simulink model "rfsoc4x2_ospfb_128"  (R2021a)
settings: Solver=VariableStepAuto  StartTime=0.0  StopTime=2048  RelTol=1e-3
undefined symbols (not defined in the file): pfb_coeff_gen_calc
libraries: xbsIndex_r4 x25898, casper_library_delays x113, casper_library_misc x68, xps_library x1
(part 83 of 221)

== system rfsoc4x2_ospfb_128/fft_wideband_real/fft_unscrambler/reorder/buf5 ==
  addr : Inport
  din : Inport  Port=2
  we : Inport  Port=3
  bram0 : xbsIndex_r4/Single Port RAM  depth=16  initVector=getfield(get_param(gcb, 'UserData'), 'initVector')  distributed_mem=Block RAM  write_mode=Read Before Write  rst=off  init_reg=0  en=off  optimize_latency=off  latency=3  optimize=Speed  dbl_ovrd=off  simulation_type=fast_sim  block_type=spram
  ddin : xbsIndex_r4/Delay  rst=off  infoeditControl=Selection of Reset will increase slice count due to use of real FFs and instead of SRLs  en=off  latency=0  reg_retiming=on  dbl_ovrd=off  block_type=delay
  debus_addr : Subsystem  AncestorBlock=casper_library_flow_control/bus_expand  mask(bus_expand){mode=divisions of equal size, outputNum=1, outputWidth=4, outputBinaryPt=0, outputArithmeticType=0, show_format=on, outputToWorkspace=off, variablePrefix=, outputToModelAsWell=on}
      mask prompts: outputNum "Number of outputs:"; outputWidth "Output width:"; outputBinaryPt "Output binary point position:"; outputArithmeticType "Output arithmetic type (ufix=0, fix=1, bool=2):"; show_format "Print format string?"; outputToWorkspace "Output to workspace?"; variablePrefix "Variable name prefix:"; outputToModelAsWell "Output to model as well?"
      mask help:
      | Expands a 'bus' made using a bus_create or Xilinx
      | concat block.
      | The input will be divided into the specified number
      | of outputs with the specified arithmetic types.
      | Divisions are made from most significant bit.
      mask init: same as rfsoc4x2_ospfb_128/bus_expand
      settings: AttributesFormatString=1 outputs: uf4.0,
      mask TypeOptions mode: divisions of equal size | divisions of arbitrary size
      mask Callback mode: %bus_expand_callback();
      mask Callback outputWidth: %bus_expand_callback();
      mask Callback outputToWorkspace: %bus_expand_callback();
  debus_din : Subsystem  AncestorBlock=casper_library_flow_control/bus_expand  mask(bus_expand){mode=divisions of arbitrary size, outputNum=2, outputWidth=36, outputBinaryPt=0, outputArithmeticType=0, show_format=on, outputToWorkspace=off, variablePrefix=, outputToModelAsWell=on}
      mask prompts: outputNum "Number of outputs:"; outputWidth "Output width:"; outputBinaryPt "Output binary point position:"; outputArithmeticType "Output arithmetic type (ufix=0, fix=1, bool=2):"; show_format "Print format string?"; outputToWorkspace "Output to workspace?"; variablePrefix "Variable name prefix:"; outputToModelAsWell "Output to model as well?"
      mask help:
      | Expands a 'bus' made using a bus_create or Xilinx
      | concat block.
      | The input will be divided into the specified number
      | of outputs with the specified arithmetic types.
      | Divisions are made from most significant bit.
      mask init: same as rfsoc4x2_ospfb_128/bus_expand
      settings: AttributesFormatString=1 outputs: uf36.0,
      mask TypeOptions mode: divisions of equal size | divisions of arbitrary size
      mask Callback mode: %bus_expand_callback();
      mask Callback outputWidth: %bus_expand_callback();
      mask Callback outputToWorkspace: %bus_expand_callback();
  debus_we : Subsystem  AncestorBlock=casper_library_flow_control/bus_expand  mask(bus_expand){mode=divisions of equal size, outputNum=1, outputWidth=1, outputBinaryPt=0, outputArithmeticType=2, show_format=on, outputToWorkspace=off, variablePrefix=, outputToModelAsWell=on}
      mask prompts: outputNum "Number of outputs:"; outputWidth "Output width:"; outputBinaryPt "Output binary point position:"; outputArithmeticType "Output arithmetic type (ufix=0, fix=1, bool=2):"; show_format "Print format string?"; outputToWorkspace "Output to workspace?"; variablePrefix "Variable name prefix:"; outputToModelAsWell "Output to model as well?"
      mask help:
      | Expands a 'bus' made using a bus_create or Xilinx
      | concat block.
      | The input will be divided into the specified number
      | of outputs with the specified arithmetic types.
      | Divisions are made from most significant bit.
      mask init: same as rfsoc4x2_ospfb_128/bus_expand
      settings: AttributesFormatString=1 outputs: b,
      mask TypeOptions mode: divisions of equal size | divisions of arbitrary size
      mask Callback mode: %bus_expand_callback();
      mask Callback outputWidth: %bus_expand_callback();
      mask Callback outputToWorkspace: %bus_expand_callback();
  din_bussify : Subsystem  AncestorBlock=casper_library_flow_control/bus_create  mask(bus_create){inputNum=1}
      mask prompts: inputNum "Number of inputs:"
      mask init:
      | bus_create_init(gcb,...
      |     'inputNum', inputNum);
  rep_addr : Subsystem  AncestorBlock=casper_library_bus/bus_replicate  mask(bus_replicate){replication=1, csp_latency=0, misc=off, implementation=core}
      mask prompts: replication "replication factor"; csp_latency "latency"; misc "misc support"; implementation "delay implementation"
      mask help: Output bus formed by replicating input bus a number of times
      mask init:
      | bus_replicate_init(gcb, ...
      |     'replication', replication, ...
      |     'csp_latency', csp_latency, ...
      |     'implementation', implementation, ...
      |     'misc', misc);
      mask TypeOptions implementation: core | behavioral
  rep_we : Subsystem  AncestorBlock=casper_library_bus/bus_replicate  mask(bus_replicate){replication=1, csp_latency=0, misc=off, implementation=core}
      mask prompts: replication "replication factor"; csp_latency "latency"; misc "misc support"; implementation "delay implementation"
      mask help: Output bus formed by replicating input bus a number of times
      mask init:
      | bus_replicate_init(gcb, ...
      |     'replication', replication, ...
      |     'csp_latency', csp_latency, ...
      |     'implementation', implementation, ...
      |     'misc', misc);
      mask TypeOptions implementation: core | behavioral
  dout : Outport
  wires:
  addr/1 -> rep_addr/1(in)
  din/1 -> ddin/1
  we/1 -> rep_we/1(in)
  rep_addr/1(out) -> debus_addr/1(bus_in)
  ddin/1 -> debus_din/1(bus_in)
  rep_we/1(out) -> debus_we/1(bus_in)
  debus_addr/1(msb_lsb_out1) -> bram0/1
  debus_din/1(msb_lsb_out1) -> bram0/2
  debus_we/1(msb_lsb_out1) -> bram0/3
  bram0/1 -> din_bussify/1(in1)
  din_bussify/1(bus_out) -> dout/1

== system rfsoc4x2_ospfb_128/fft_wideband_real/fft_unscrambler/reorder/buf6 ==
  addr : Inport
  din : Inport  Port=2
  we : Inport  Port=3
  bram0 : xbsIndex_r4/Single Port RAM  depth=16  initVector=getfield(get_param(gcb, 'UserData'), 'initVector')  distributed_mem=Block RAM  write_mode=Read Before Write  rst=off  init_reg=0  en=off  optimize_latency=off  latency=3  optimize=Speed  dbl_ovrd=off  simulation_type=fast_sim  block_type=spram
  ddin : xbsIndex_r4/Delay  rst=off  infoeditControl=Selection of Reset will increase slice count due to use of real FFs and instead of SRLs  en=off  latency=0  reg_retiming=on  dbl_ovrd=off  block_type=delay
  debus_addr : Subsystem  AncestorBlock=casper_library_flow_control/bus_expand  mask(bus_expand){mode=divisions of equal size, outputNum=1, outputWidth=4, outputBinaryPt=0, outputArithmeticType=0, show_format=on, outputToWorkspace=off, variablePrefix=, outputToModelAsWell=on}
      mask prompts: outputNum "Number of outputs:"; outputWidth "Output width:"; outputBinaryPt "Output binary point position:"; outputArithmeticType "Output arithmetic type (ufix=0, fix=1, bool=2):"; show_format "Print format string?"; outputToWorkspace "Output to workspace?"; variablePrefix "Variable name prefix:"; outputToModelAsWell "Output to model as well?"
      mask help:
      | Expands a 'bus' made using a bus_create or Xilinx
      | concat block.
      | The input will be divided into the specified number
      | of outputs with the specified arithmetic types.
      | Divisions are made from most significant bit.
      mask init: same as rfsoc4x2_ospfb_128/bus_expand
      settings: AttributesFormatString=1 outputs: uf4.0,
      mask TypeOptions mode: divisions of equal size | divisions of arbitrary size
      mask Callback mode: %bus_expand_callback();
      mask Callback outputWidth: %bus_expand_callback();
      mask Callback outputToWorkspace: %bus_expand_callback();
  debus_din : Subsystem  AncestorBlock=casper_library_flow_control/bus_expand  mask(bus_expand){mode=divisions of arbitrary size, outputNum=2, outputWidth=36, outputBinaryPt=0, outputArithmeticType=0, show_format=on, outputToWorkspace=off, variablePrefix=, outputToModelAsWell=on}
      mask prompts: outputNum "Number of outputs:"; outputWidth "Output width:"; outputBinaryPt "Output binary point position:"; outputArithmeticType "Output arithmetic type (ufix=0, fix=1, bool=2):"; show_format "Print format string?"; outputToWorkspace "Output to workspace?"; variablePrefix "Variable name prefix:"; outputToModelAsWell "Output to model as well?"
      mask help:
      | Expands a 'bus' made using a bus_create or Xilinx
      | concat block.
      | The input will be divided into the specified number
      | of outputs with the specified arithmetic types.
      | Divisions are made from most significant bit.
      mask init: same as rfsoc4x2_ospfb_128/bus_expand
      settings: AttributesFormatString=1 outputs: uf36.0,
      mask TypeOptions mode: divisions of equal size | divisions of arbitrary size
      mask Callback mode: %bus_expand_callback();
      mask Callback outputWidth: %bus_expand_callback();
      mask Callback outputToWorkspace: %bus_expand_callback();
  debus_we : Subsystem  AncestorBlock=casper_library_flow_control/bus_expand  mask(bus_expand){mode=divisions of equal size, outputNum=1, outputWidth=1, outputBinaryPt=0, outputArithmeticType=2, show_format=on, outputToWorkspace=off, variablePrefix=, outputToModelAsWell=on}
      mask prompts: outputNum "Number of outputs:"; outputWidth "Output width:"; outputBinaryPt "Output binary point position:"; outputArithmeticType "Output arithmetic type (ufix=0, fix=1, bool=2):"; show_format "Print format string?"; outputToWorkspace "Output to workspace?"; variablePrefix "Variable name prefix:"; outputToModelAsWell "Output to model as well?"
      mask help:
      | Expands a 'bus' made using a bus_create or Xilinx
      | concat block.
      | The input will be divided into the specified number
      | of outputs with the specified arithmetic types.
      | Divisions are made from most significant bit.
      mask init: same as rfsoc4x2_ospfb_128/bus_expand
      settings: AttributesFormatString=1 outputs: b,
      mask TypeOptions mode: divisions of equal size | divisions of arbitrary size
      mask Callback mode: %bus_expand_callback();
      mask Callback outputWidth: %bus_expand_callback();
      mask Callback outputToWorkspace: %bus_expand_callback();
  din_bussify : Subsystem  AncestorBlock=casper_library_flow_control/bus_create  mask(bus_create){inputNum=1}
      mask prompts: inputNum "Number of inputs:"
      mask init:
      | bus_create_init(gcb,...
      |     'inputNum', inputNum);
  rep_addr : Subsystem  AncestorBlock=casper_library_bus/bus_replicate  mask(bus_replicate){replication=1, csp_latency=0, misc=off, implementation=core}
      mask prompts: replication "replication factor"; csp_latency "latency"; misc "misc support"; implementation "delay implementation"
      mask help: Output bus formed by replicating input bus a number of times
      mask init:
      | bus_replicate_init(gcb, ...
      |     'replication', replication, ...
      |     'csp_latency', csp_latency, ...
      |     'implementation', implementation, ...
      |     'misc', misc);
      mask TypeOptions implementation: core | behavioral
  rep_we : Subsystem  AncestorBlock=casper_library_bus/bus_replicate  mask(bus_replicate){replication=1, csp_latency=0, misc=off, implementation=core}
      mask prompts: replication "replication factor"; csp_latency "latency"; misc "misc support"; implementation "delay implementation"
      mask help: Output bus formed by replicating input bus a number of times
      mask init:
      | bus_replicate_init(gcb, ...
      |     'replication', replication, ...
      |     'csp_latency', csp_latency, ...
      |     'implementation', implementation, ...
      |     'misc', misc);
      mask TypeOptions implementation: core | behavioral
  dout : Outport
  wires:
  addr/1 -> rep_addr/1(in)
  din/1 -> ddin/1
  we/1 -> rep_we/1(in)
  rep_addr/1(out) -> debus_addr/1(bus_in)
  ddin/1 -> debus_din/1(bus_in)
  rep_we/1(out) -> debus_we/1(bus_in)
  debus_addr/1(msb_lsb_out1) -> bram0/1
  debus_din/1(msb_lsb_out1) -> bram0/2
  debus_we/1(msb_lsb_out1) -> bram0/3
  bram0/1 -> din_bussify/1(in1)
  din_bussify/1(bus_out) -> dout/1

== system rfsoc4x2_ospfb_128/fft_wideband_real/fft_unscrambler/reorder/buf7 ==
  addr : Inport
  din : Inport  Port=2
  we : Inport  Port=3
  bram0 : xbsIndex_r4/Single Port RAM  depth=16  initVector=getfield(get_param(gcb, 'UserData'), 'initVector')  distributed_mem=Block RAM  write_mode=Read Before Write  rst=off  init_reg=0  en=off  optimize_latency=off  latency=3  optimize=Speed  dbl_ovrd=off  simulation_type=fast_sim  block_type=spram
  ddin : xbsIndex_r4/Delay  rst=off  infoeditControl=Selection of Reset will increase slice count due to use of real FFs and instead of SRLs  en=off  latency=0  reg_retiming=on  dbl_ovrd=off  block_type=delay
  debus_addr : Subsystem  AncestorBlock=casper_library_flow_control/bus_expand  mask(bus_expand){mode=divisions of equal size, outputNum=1, outputWidth=4, outputBinaryPt=0, outputArithmeticType=0, show_format=on, outputToWorkspace=off, variablePrefix=, outputToModelAsWell=on}
      mask prompts: outputNum "Number of outputs:"; outputWidth "Output width:"; outputBinaryPt "Output binary point position:"; outputArithmeticType "Output arithmetic type (ufix=0, fix=1, bool=2):"; show_format "Print format string?"; outputToWorkspace "Output to workspace?"; variablePrefix "Variable name prefix:"; outputToModelAsWell "Output to model as well?"
      mask help:
      | Expands a 'bus' made using a bus_create or Xilinx
      | concat block.
      | The input will be divided into the specified number
      | of outputs with the specified arithmetic types.
      | Divisions are made from most significant bit.
      mask init: same as rfsoc4x2_ospfb_128/bus_expand
      settings: AttributesFormatString=1 outputs: uf4.0,
      mask TypeOptions mode: divisions of equal size | divisions of arbitrary size
      mask Callback mode: %bus_expand_callback();
      mask Callback outputWidth: %bus_expand_callback();
      mask Callback outputToWorkspace: %bus_expand_callback();
  debus_din : Subsystem  AncestorBlock=casper_library_flow_control/bus_expand  mask(bus_expand){mode=divisions of arbitrary size, outputNum=2, outputWidth=36, outputBinaryPt=0, outputArithmeticType=0, show_format=on, outputToWorkspace=off, variablePrefix=, outputToModelAsWell=on}
      mask prompts: outputNum "Number of outputs:"; outputWidth "Output width:"; outputBinaryPt "Output binary point position:"; outputArithmeticType "Output arithmetic type (ufix=0, fix=1, bool=2):"; show_format "Print format string?"; outputToWorkspace "Output to workspace?"; variablePrefix "Variable name prefix:"; outputToModelAsWell "Output to model as well?"
      mask help:
      | Expands a 'bus' made using a bus_create or Xilinx
      | concat block.
      | The input will be divided into the specified number
      | of outputs with the specified arithmetic types.
      | Divisions are made from most significant bit.
      mask init: same as rfsoc4x2_ospfb_128/bus_expand
      settings: AttributesFormatString=1 outputs: uf36.0,
      mask TypeOptions mode: divisions of equal size | divisions of arbitrary size
      mask Callback mode: %bus_expand_callback();
      mask Callback outputWidth: %bus_expand_callback();
      mask Callback outputToWorkspace: %bus_expand_callback();
  debus_we : Subsystem  AncestorBlock=casper_library_flow_control/bus_expand  mask(bus_expand){mode=divisions of equal size, outputNum=1, outputWidth=1, outputBinaryPt=0, outputArithmeticType=2, show_format=on, outputToWorkspace=off, variablePrefix=, outputToModelAsWell=on}
      mask prompts: outputNum "Number of outputs:"; outputWidth "Output width:"; outputBinaryPt "Output binary point position:"; outputArithmeticType "Output arithmetic type (ufix=0, fix=1, bool=2):"; show_format "Print format string?"; outputToWorkspace "Output to workspace?"; variablePrefix "Variable name prefix:"; outputToModelAsWell "Output to model as well?"
      mask help:
      | Expands a 'bus' made using a bus_create or Xilinx
      | concat block.
      | The input will be divided into the specified number
      | of outputs with the specified arithmetic types.
      | Divisions are made from most significant bit.
      mask init: same as rfsoc4x2_ospfb_128/bus_expand
      settings: AttributesFormatString=1 outputs: b,
      mask TypeOptions mode: divisions of equal size | divisions of arbitrary size
      mask Callback mode: %bus_expand_callback();
      mask Callback outputWidth: %bus_expand_callback();
      mask Callback outputToWorkspace: %bus_expand_callback();
  din_bussify : Subsystem  AncestorBlock=casper_library_flow_control/bus_create  mask(bus_create){inputNum=1}
      mask prompts: inputNum "Number of inputs:"
      mask init:
      | bus_create_init(gcb,...
      |     'inputNum', inputNum);
  rep_addr : Subsystem  AncestorBlock=casper_library_bus/bus_replicate  mask(bus_replicate){replication=1, csp_latency=0, misc=off, implementation=core}
      mask prompts: replication "replication factor"; csp_latency "latency"; misc "misc support"; implementation "delay implementation"
      mask help: Output bus formed by replicating input bus a number of times
      mask init:
      | bus_replicate_init(gcb, ...
      |     'replication', replication, ...
      |     'csp_latency', csp_latency, ...
      |     'implementation', implementation, ...
      |     'misc', misc);
      mask TypeOptions implementation: core | behavioral
  rep_we : Subsystem  AncestorBlock=casper_library_bus/bus_replicate  mask(bus_replicate){replication=1, csp_latency=0, misc=off, implementation=core}
      mask prompts: replication "replication factor"; csp_latency "latency"; misc "misc support"; implementation "delay implementation"
      mask help: Output bus formed by replicating input bus a number of times
      mask init:
      | bus_replicate_init(gcb, ...
      |     'replication', replication, ...
      |     'csp_latency', csp_latency, ...
      |     'implementation', implementation, ...
      |     'misc', misc);
      mask TypeOptions implementation: core | behavioral
  dout : Outport
  wires:
  addr/1 -> rep_addr/1(in)
  din/1 -> ddin/1
  we/1 -> rep_we/1(in)
  rep_addr/1(out) -> debus_addr/1(bus_in)
  ddin/1 -> debus_din/1(bus_in)
  rep_we/1(out) -> debus_we/1(bus_in)
  debus_addr/1(msb_lsb_out1) -> bram0/1
  debus_din/1(msb_lsb_out1) -> bram0/2
  debus_we/1(msb_lsb_out1) -> bram0/3
  bram0/1 -> din_bussify/1(in1)
  din_bussify/1(bus_out) -> dout/1

== system rfsoc4x2_ospfb_128/fft_wideband_real/fft_unscrambler/reorder/current_map ==
  addra : Inport
  dina : Inport  Port=2
  wea : Inport  Port=3
  addrb : Inport  Port=4
  dinb : Inport  Port=5
  web : Inport  Port=6
  A_bussify0 : Subsystem  AncestorBlock=casper_library_flow_control/bus_create  mask(bus_create){inputNum=1}
      mask prompts: inputNum "Number of inputs:"
      mask init:
      | bus_create_init(gcb,...
      |     'inputNum', inputNum);
  B_bussify0 : Subsystem  AncestorBlock=casper_library_flow_control/bus_create  mask(bus_create){inputNum=1}
      mask prompts: inputNum "Number of inputs:"
      mask init:
      | bus_create_init(gcb,...
      |     'inputNum', inputNum);
  alsbs_slice : xbsIndex_r4/Slice  nbits=4  boolean_output=off  mode=Lower Bit Location + Width  bit1=0  base1=LSB of Input  bit0=0  base0=LSB of Input  dbl_ovrd=off  block_type=slice
  blsbs_slice : xbsIndex_r4/Slice  nbits=4  boolean_output=off  mode=Lower Bit Location + Width  bit1=0  base1=LSB of Input  bit0=0  base0=LSB of Input  dbl_ovrd=off  block_type=slice
  bram0_0 : xbsIndex_r4/Dual Port RAM  depth=16  initVector=getfield(get_param(gcb, 'UserData'), 'initVector')  distributed_mem=Block RAM  init_a=0  init_b=0  rst_a=off  rst_b=off  en_a=off  en_b=off  latency=2  write_mode_A=Read Before Write  write_mode_B=Read Before Write  optimize=Speed  dbl_ovrd=off  simulation_type=fast_sim  block_type=dpram
  ddina0 : xbsIndex_r4/Delay  rst=off  infoeditControl=Selection of Reset will increase slice count due to use of real FFs and instead of SRLs  en=off  latency=0  reg_retiming=on  dbl_ovrd=off  block_type=delay
  ddinb0 : xbsIndex_r4/Delay  rst=off  infoeditControl=Selection of Reset will increase slice count due to use of real FFs and instead of SRLs  en=off  latency=0  reg_retiming=on  dbl_ovrd=off  block_type=delay
  debus_addra0 : Subsystem  AncestorBlock=casper_library_flow_control/bus_expand  mask(bus_expand){mode=divisions of equal size, outputNum=1, outputWidth=4, outputBinaryPt=0, outputArithmeticType=0, show_format=on, outputToWorkspace=off, variablePrefix=, outputToModelAsWell=on}
      mask prompts: outputNum "Number of outputs:"; outputWidth "Output width:"; outputBinaryPt "Output binary point position:"; outputArithmeticType "Output arithmetic type (ufix=0, fix=1, bool=2):"; show_format "Print format string?"; outputToWorkspace "Output to workspace?"; variablePrefix "Variable name prefix:"; outputToModelAsWell "Output to model as well?"
      mask help:
      | Expands a 'bus' made using a bus_create or Xilinx
      | concat block.
      | The input will be divided into the specified number
      | of outputs with the specified arithmetic types.
      | Divisions are made from most significant bit.
      mask init: same as rfsoc4x2_ospfb_128/bus_expand
      settings: AttributesFormatString=1 outputs: uf4.0,
      mask TypeOptions mode: divisions of equal size | divisions of arbitrary size
      mask Callback mode: %bus_expand_callback();
      mask Callback outputWidth: %bus_expand_callback();
      mask Callback outputToWorkspace: %bus_expand_callback();
  debus_addrb0 : Subsystem  AncestorBlock=casper_library_flow_control/bus_expand  mask(bus_expand){mode=divisions of equal size, outputNum=1, outputWidth=4, outputBinaryPt=0, outputArithmeticType=0, show_format=on, outputToWorkspace=off, variablePrefix=, outputToModelAsWell=on}
      mask prompts: outputNum "Number of outputs:"; outputWidth "Output width:"; outputBinaryPt "Output binary point position:"; outputArithmeticType "Output arithmetic type (ufix=0, fix=1, bool=2):"; show_format "Print format string?"; outputToWorkspace "Output to workspace?"; variablePrefix "Variable name prefix:"; outputToModelAsWell "Output to model as well?"
      mask help:
      | Expands a 'bus' made using a bus_create or Xilinx
      | concat block.
      | The input will be divided into the specified number
      | of outputs with the specified arithmetic types.
      | Divisions are made from most significant bit.
      mask init: same as rfsoc4x2_ospfb_128/bus_expand
      settings: AttributesFormatString=1 outputs: uf4.0,
      mask TypeOptions mode: divisions of equal size | divisions of arbitrary size
      mask Callback mode: %bus_expand_callback();
      mask Callback outputWidth: %bus_expand_callback();
      mask Callback outputToWorkspace: %bus_expand_callback();
  debus_dina0 : Subsystem  AncestorBlock=casper_library_flow_control/bus_expand  mask(bus_expand){mode=divisions of arbitrary size, outputNum=2, outputWidth=4, outputBinaryPt=0, outputArithmeticType=0, show_format=on, outputToWorkspace=off, variablePrefix=, outputToModelAsWell=on}
      mask prompts: outputNum "Number of outputs:"; outputWidth "Output width:"; outputBinaryPt "Output binary point position:"; outputArithmeticType "Output arithmetic type (ufix=0, fix=1, bool=2):"; show_format "Print format string?"; outputToWorkspace "Output to workspace?"; variablePrefix "Variable name prefix:"; outputToModelAsWell "Output to model as well?"
      mask help:
      | Expands a 'bus' made using a bus_create or Xilinx
      | concat block.
      | The input will be divided into the specified number
      | of outputs with the specified arithmetic types.
      | Divisions are made from most significant bit.
      mask init: same as rfsoc4x2_ospfb_128/bus_expand
      settings: AttributesFormatString=1 outputs: uf4.0,
      mask TypeOptions mode: divisions of equal size | divisions of arbitrary size
      mask Callback mode: %bus_expand_callback();
      mask Callback outputWidth: %bus_expand_callback();
      mask Callback outputToWorkspace: %bus_expand_callback();
  debus_dinb0 : Subsystem  AncestorBlock=casper_library_flow_control/bus_expand  mask(bus_expand){mode=divisions of arbitrary size, outputNum=2, outputWidth=4, outputBinaryPt=0, outputArithmeticType=0, show_format=on, outputToWorkspace=off, variablePrefix=, outputToModelAsWell=on}
      mask prompts: outputNum "Number of outputs:"; outputWidth "Output width:"; outputBinaryPt "Output binary point position:"; outputArithmeticType "Output arithmetic type (ufix=0, fix=1, bool=2):"; show_format "Print format string?"; outputToWorkspace "Output to workspace?"; variablePrefix "Variable name prefix:"; outputToModelAsWell "Output to model as well?"
      mask help:
      | Expands a 'bus' made using a bus_create or Xilinx
      | concat block.
      | The input will be divided into the specified number
      | of outputs with the specified arithmetic types.
      | Divisions are made from most significant bit.
      mask init: same as rfsoc4x2_ospfb_128/bus_expand
      settings: AttributesFormatString=1 outputs: uf4.0,
      mask TypeOptions mode: divisions of equal size | divisions of arbitrary size
      mask Callback mode: %bus_expand_callback();
      mask Callback outputWidth: %bus_expand_callback();
      mask Callback outputToWorkspace: %bus_expand_callback();
  debus_wea0 : Subsystem  AncestorBlock=casper_library_flow_control/bus_expand  mask(bus_expand){mode=divisions of equal size, outputNum=1, outputWidth=1, outputBinaryPt=0, outputArithmeticType=2, show_format=on, outputToWorkspace=off, variablePrefix=, outputToModelAsWell=on}
      mask prompts: outputNum "Number of outputs:"; outputWidth "Output width:"; outputBinaryPt "Output binary point position:"; outputArithmeticType "Output arithmetic type (ufix=0, fix=1, bool=2):"; show_format "Print format string?"; outputToWorkspace "Output to workspace?"; variablePrefix "Variable name prefix:"; outputToModelAsWell "Output to model as well?"
      mask help:
      | Expands a 'bus' made using a bus_create or Xilinx
      | concat block.
      | The input will be divided into the specified number
      | of outputs with the specified arithmetic types.
      | Divisions are made from most significant bit.
      mask init: same as rfsoc4x2_ospfb_128/bus_expand
      settings: AttributesFormatString=1 outputs: b,
      mask TypeOptions mode: divisions of equal size | divisions of arbitrary size
      mask Callback mode: %bus_expand_callback();
      mask Callback outputWidth: %bus_expand_callback();
      mask Callback outputToWorkspace: %bus_expand_callback();
  debus_web0 : Subsystem  AncestorBlock=casper_library_flow_control/bus_expand  mask(bus_expand){mode=divisions of equal size, outputNum=1, outputWidth=1, outputBinaryPt=0, outputArithmeticType=2, show_format=on, outputToWorkspace=off, variablePrefix=, outputToModelAsWell=on}
      mask prompts: outputNum "Number of outputs:"; outputWidth "Output width:"; outputBinaryPt "Output binary point position:"; outputArithmeticType "Output arithmetic type (ufix=0, fix=1, bool=2):"; show_format "Print format string?"; outputToWorkspace "Output to workspace?"; variablePrefix "Variable name prefix:"; outputToModelAsWell "Output to model as well?"
      mask help:
      | Expands a 'bus' made using a bus_create or Xilinx
      | concat block.
      | The input will be divided into the specified number
      | of outputs with the specified arithmetic types.
      | Divisions are made from most significant bit.
      mask init: same as rfsoc4x2_ospfb_128/bus_expand
      settings: AttributesFormatString=1 outputs: b,
      mask TypeOptions mode: divisions of equal size | divisions of arbitrary size
      mask Callback mode: %bus_expand_callback();
      mask Callback outputWidth: %bus_expand_callback();
      mask Callback outputToWorkspace: %bus_expand_callback();
  rep_addra0 : Subsystem  AncestorBlock=casper_library_bus/bus_replicate  mask(bus_replicate){replication=1, csp_latency=4, misc=off, implementation=behavioral}
      mask prompts: replication "replication factor"; csp_latency "latency"; misc "misc support"; implementation "delay implementation"
      mask help: Output bus formed by replicating input bus a number of times
      mask init:
      | bus_replicate_init(gcb, ...
      |     'replication', replication, ...
      |     'csp_latency', csp_latency, ...
      |     'implementation', implementation, ...
      |     'misc', misc);
      mask TypeOptions implementation: core | behavioral
  rep_addrb0 : Subsystem  AncestorBlock=casper_library_bus/bus_replicate  mask(bus_replicate){replication=1, csp_latency=0, misc=off, implementation=core}
      mask prompts: replication "replication factor"; csp_latency "latency"; misc "misc support"; implementation "delay implementation"
      mask help: Output bus formed by replicating input bus a number of times
      mask init:
      | bus_replicate_init(gcb, ...
      |     'replication', replication, ...
      |     'csp_latency', csp_latency, ...
      |     'implementation', implementation, ...
      |     'misc', misc);
      mask TypeOptions implementation: core | behavioral
  rep_wea0 : Subsystem  AncestorBlock=casper_library_bus/bus_replicate  mask(bus_replicate){replication=1, csp_latency=4, misc=off, implementation=core}
      mask prompts: replication "replication factor"; csp_latency "latency"; misc "misc support"; implementation "delay implementation"
      mask help: Output bus formed by replicating input bus a number of times
      mask init:
      | bus_replicate_init(gcb, ...
      |     'replication', replication, ...
      |     'csp_latency', csp_latency, ...
      |     'implementation', implementation, ...
      |     'misc', misc);
      mask TypeOptions implementation: core | behavioral
  rep_web0 : Subsystem  AncestorBlock=casper_library_bus/bus_replicate  mask(bus_replicate){replication=1, csp_latency=0, misc=off, implementation=behavioral}
      mask prompts: replication "replication factor"; csp_latency "latency"; misc "misc support"; implementation "delay implementation"
      mask help: Output bus formed by replicating input bus a number of times
      mask init:
      | bus_replicate_init(gcb, ...
      |     'replication', replication, ...
      |     'csp_latency', csp_latency, ...
      |     'implementation', implementation, ...
      |     'misc', misc);
      mask TypeOptions implementation: core | behavioral
  A : Outport
  B : Outport  Port=2
  wires:
  addrb/1 -> blsbs_slice/1
  addra/1 -> alsbs_slice/1
  blsbs_slice/1 -> rep_addrb0/1(in)
  alsbs_slice/1 -> rep_addra0/1(in)
  dina/1 -> ddina0/1
  wea/1 -> rep_wea0/1(in)
  dinb/1 -> ddinb0/1
  web/1 -> rep_web0/1(in)
  rep_addrb0/1(out) -> debus_addrb0/1(bus_in)
  rep_addra0/1(out) -> debus_addra0/1(bus_in)
  ddina0/1 -> debus_dina0/1(bus_in)
  rep_wea0/1(out) -> debus_wea0/1(bus_in)
  ddinb0/1 -> debus_dinb0/1(bus_in)
  rep_web0/1(out) -> debus_web0/1(bus_in)
  debus_addra0/1(msb_lsb_out1) -> bram0_0/1
  debus_dina0/1(msb_lsb_out1) -> bram0_0/2
  debus_wea0/1(msb_lsb_out1) -> bram0_0/3
  debus_addrb0/1(msb_lsb_out1) -> bram0_0/4
  debus_dinb0/1(msb_lsb_out1) -> bram0_0/5
  debus_web0/1(msb_lsb_out1) -> bram0_0/6
  bram0_0/1 -> A_bussify0/1(in1)
  bram0_0/2 -> B_bussify0/1(in1)
  A_bussify0/1(bus_out) -> A/1
  B_bussify0/1(bus_out) -> B/1

== system rfsoc4x2_ospfb_128/fft_wideband_real/fft_unscrambler/reorder/edge_detect ==
  in : Inport
  Delay : xbsIndex_r4/Delay  rst=off  infoeditControl=Selection of Reset will increase slice count due to use of real FFs and instead of SRLs  en=off  latency=1  reg_retiming=off  dbl_ovrd=off  block_type=delay
      settings: xl_area=[0, 0, 0, 0, 0, 0, 0]
  Inverter : xbsIndex_r4/Inverter  en=off  latency=0  dbl_ovrd=off  block_type=inv
      settings: xl_area=[0, 0, 0, 0, 0, 0, 0]
  edge_op : xbsIndex_r4/Logical  logical_function=AND  inputs=2  en=off  latency=0  precision=Full  arith_type=Unsigned  n_bits=8  bin_pt=2  align_bp=on  dbl_ovrd=off  block_type=logical
      settings: xl_area=[0, 0, 0, 0, 0, 0, 0]
  out : Outport  VectorParamsAs1DForOutWhenUnconnected=off
  wires:
  Inverter/1 -> edge_op/1
  edge_op/1 -> out/1
  in/1 -> Inverter/1, Delay/1
  Delay/1 -> edge_op/2

== system rfsoc4x2_ospfb_128/fft_wideband_real/fft_unscrambler/reorder/we_expand ==
  bus_in : Inport
  slice1 : xbsIndex_r4/Slice  nbits=1  boolean_output=on  mode=Upper Bit Location + Width  bit1=-7  base1=MSB of Input  bit0=0  base0=LSB of Input  dbl_ovrd=off  block_type=slice
  slice2 : xbsIndex_r4/Slice  nbits=1  boolean_output=on  mode=Upper Bit Location + Width  bit1=-6  base1=MSB of Input  bit0=0  base0=LSB of Input  dbl_ovrd=off  block_type=slice
  slice3 : xbsIndex_r4/Slice  nbits=1  boolean_output=on  mode=Upper Bit Location + Width  bit1=-5  base1=MSB of Input  bit0=0  base0=LSB of Input  dbl_ovrd=off  block_type=slice
  slice4 : xbsIndex_r4/Slice  nbits=1  boolean_output=on  mode=Upper Bit Location + Width  bit1=-4  base1=MSB of Input  bit0=0  base0=LSB of Input  dbl_ovrd=off  block_type=slice
  slice5 : xbsIndex_r4/Slice  nbits=1  boolean_output=on  mode=Upper Bit Location + Width  bit1=-3  base1=MSB of Input  bit0=0  base0=LSB of Input  dbl_ovrd=off  block_type=slice
  slice6 : xbsIndex_r4/Slice  nbits=1  boolean_output=on  mode=Upper Bit Location + Width  bit1=-2  base1=MSB of Input  bit0=0  base0=LSB of Input  dbl_ovrd=off  block_type=slice
  slice7 : xbsIndex_r4/Slice  nbits=1  boolean_output=on  mode=Upper Bit Location + Width  bit1=-1  base1=MSB of Input  bit0=0  base0=LSB of Input  dbl_ovrd=off  block_type=slice
  slice8 : xbsIndex_r4/Slice  nbits=1  boolean_output=on  mode=Upper Bit Location + Width  bit1=0  base1=MSB of Input  bit0=0  base0=LSB of Input  dbl_ovrd=off  block_type=slice
  msb_out8 : Outport
  out7 : Outport  Port=2
  out6 : Outport  Port=3
  out5 : Outport  Port=4
  out4 : Outport  Port=5
  out3 : Outport  Port=6
  out2 : Outport  Port=7
  lsb_out1 : Outport  Port=8  VectorParamsAs1DForOutWhenUnconnected=off
  wires:
  bus_in/1 -> slice8/1, slice7/1, slice6/1, slice5/1, slice4/1, slice3/1, slice2/1, slice1/1
  slice8/1 -> msb_out8/1
  slice7/1 -> out7/1
  slice6/1 -> out6/1
  slice5/1 -> out5/1
  slice4/1 -> out4/1
  slice3/1 -> out3/1
  slice2/1 -> out2/1
  slice1/1 -> lsb_out1/1

== system rfsoc4x2_ospfb_128/fft_wideband_real/fft_unscrambler/reorder/we_replicate ==
  in : Inport
  bussify : Subsystem  AncestorBlock=casper_library_flow_control/bus_create  mask(bus_create){inputNum=8}
      mask prompts: inputNum "Number of inputs:"
      mask init:
      | bus_create_init(gcb,...
      |     'inputNum', inputNum);
  din0_0 : xbsIndex_r4/Delay  rst=off  infoeditControl=Selection of Reset will increase slice count due to use of real FFs and instead of SRLs  en=off  latency=1  reg_retiming=off  dbl_ovrd=off  block_type=delay
  din0_1 : xbsIndex_r4/Delay  rst=off  infoeditControl=Selection of Reset will increase slice count due to use of real FFs and instead of SRLs  en=off  latency=1  reg_retiming=off  dbl_ovrd=off  block_type=delay
  din1_{0..3} (4 alike) : xbsIndex_r4/Delay  rst=off  infoeditControl=Selection of Reset will increase slice count due to use of real FFs and instead of SRLs  en=off  latency=1  reg_retiming=off  dbl_ovrd=off  block_type=delay
  din2_{0..7} (8 alike) : xbsIndex_r4/Delay  rst=off  infoeditControl=Selection of Reset will increase slice count due to use of real FFs and instead of SRLs  en=off  latency=1  reg_retiming=off  dbl_ovrd=off  block_type=delay
  out : Outport
  wires:
  in/1 -> din0_0/1, din0_1/1
  din0_0/1 -> din1_0/1, din1_2/1
  din0_1/1 -> din1_1/1, din1_3/1
  din1_0/1 -> din2_0/1, din2_4/1
  din1_1/1 -> din2_1/1, din2_5/1
  din1_2/1 -> din2_2/1, din2_6/1
  din1_3/1 -> din2_3/1, din2_7/1
  din2_0/1 -> bussify/1(in1)
  din2_1/1 -> bussify/2(in2)
  din2_2/1 -> bussify/3(in3)
  din2_3/1 -> bussify/4(in4)
  din2_4/1 -> bussify/5(in5)
  din2_5/1 -> bussify/6(in6)
  din2_6/1 -> bussify/7(in7)
  din2_7/1 -> bussify/8(in8)
  bussify/1(bus_out) -> out/1

== system rfsoc4x2_ospfb_128/fft_wideband_real/fft_unscrambler/square_transposer/barrel_switcher ==
  sel : Inport
  sync_in : Inport  Port=2
  In1 : Inport  Port=3
  In2 : Inport  Port=4
  In3 : Inport  Port=5
  In4 : Inport  Port=6
  In5 : Inport  Port=7
  In6 : Inport  Port=8
  In7 : Inport  Port=9
  In8 : Inport  Port=10
  Delay1 : xbsIndex_r4/Delay  rst=off  infoeditControl=Selection of Reset will increase slice count due to use of real FFs and instead of SRLs  en=off  latency=1  reg_retiming=on  dbl_ovrd=off  block_type=delay
  Delay2 : xbsIndex_r4/Delay  rst=off  infoeditControl=Selection of Reset will increase slice count due to use of real FFs and instead of SRLs  en=off  latency=1  reg_retiming=on  dbl_ovrd=off  block_type=delay
  Delay_sync : xbsIndex_r4/Delay  rst=off  infoeditControl=Selection of Reset will increase slice count due to use of real FFs and instead of SRLs  en=off  latency=3  reg_retiming=on  dbl_ovrd=off  block_type=delay
  Mux{11..13,21..23,31..33,41..43,51..53,61..63,71..73,81..83} (24 alike) : xbsIndex_r4/Mux  inputs=2  en=off  latency=1  precision=Full  arith_type=Unsigned  n_bits=16  bin_pt=14  quantization=Truncate  overflow=Wrap  dbl_ovrd=off  block_type=mux
  Slice1 : xbsIndex_r4/Slice  nbits=1  boolean_output=off  mode=Upper Bit Location + Width  bit1=-0  base1=MSB of Input  bit0=0  base0=LSB of Input  dbl_ovrd=off  block_type=slice
  Slice2 : xbsIndex_r4/Slice  nbits=1  boolean_output=off  mode=Upper Bit Location + Width  bit1=-1  base1=MSB of Input  bit0=0  base0=LSB of Input  dbl_ovrd=off  block_type=slice
  Slice3 : xbsIndex_r4/Slice  nbits=1  boolean_output=off  mode=Upper Bit Location + Width  bit1=-2  base1=MSB of Input  bit0=0  base0=LSB of Input  dbl_ovrd=off  block_type=slice
  sync_out : Outport
  Out1 : Outport  Port=2
  Out2 : Outport  Port=3
  Out3 : Outport  Port=4
  Out4 : Outport  Port=5
  Out5 : Outport  Port=6
  Out6 : Outport  Port=7
  Out7 : Outport  Port=8
  Out8 : Outport  Port=9
  wires:
  sync_in/1 -> Delay_sync/1
  Delay_sync/1 -> sync_out/1
  sel/1 -> Slice1/1, Delay1/1
  Delay1/1 -> Delay2/1, Slice2/1
  Delay2/1 -> Slice3/1
  Slice1/1 -> Mux11/1, Mux21/1, Mux31/1, Mux41/1, Mux51/1, Mux61/1, Mux71/1, Mux81/1
  Slice2/1 -> Mux12/1, Mux22/1, Mux32/1, Mux42/1, Mux52/1, Mux62/1, Mux72/1, Mux82/1
  Slice3/1 -> Mux13/1, Mux23/1, Mux33/1, Mux43/1, Mux53/1, Mux63/1, Mux73/1, Mux83/1
  In1/1 -> Mux11/2, Mux51/3
  Mux13/1 -> Out1/1
  In2/1 -> Mux21/2, Mux61/3
  Mux23/1 -> Out2/1
  In3/1 -> Mux31/2, Mux71/3
  Mux33/1 -> Out3/1
  In4/1 -> Mux41/2, Mux81/3
  Mux43/1 -> Out4/1
  In5/1 -> Mux51/2, Mux11/3
  Mux53/1 -> Out5/1
  In6/1 -> Mux61/2, Mux21/3
  Mux63/1 -> Out6/1
  In7/1 -> Mux71/2, Mux31/3
  Mux73/1 -> Out7/1
  In8/1 -> Mux81/2, Mux41/3
  Mux83/1 -> Out8/1
  Mux11/1 -> Mux12/2, Mux72/3
  Mux12/1 -> Mux13/2, Mux83/3
  Mux21/1 -> Mux22/2, Mux82/3
  Mux22/1 -> Mux23/2, Mux13/3
  Mux31/1 -> Mux32/2, Mux12/3
  Mux32/1 -> Mux33/2, Mux23/3
  Mux41/1 -> Mux42/2, Mux22/3
  Mux42/1 -> Mux43/2, Mux33/3
  Mux51/1 -> Mux52/2, Mux32/3
  Mux52/1 -> Mux53/2, Mux43/3
  Mux61/1 -> Mux62/2, Mux42/3
  Mux62/1 -> Mux63/2, Mux53/3
  Mux71/1 -> Mux72/2, Mux52/3
  Mux72/1 -> Mux73/2, Mux63/3
  Mux81/1 -> Mux82/2, Mux62/3
  Mux82/1 -> Mux83/2, Mux73/3

== system rfsoc4x2_ospfb_128/fft_wideband_real/fft_unscrambler/square_transposer/db0 ==
  din : Inport
  dly : xbsIndex_r4/Delay  rst=off  infoeditControl=Selection of Reset will increase slice count due to use of real FFs and instead of SRLs  en=off  latency=DelayLen  reg_retiming=on  dbl_ovrd=off  block_type=delay
  dout : Outport
  wires:
  din/1 -> dly/1
  dly/1 -> dout/1

== system rfsoc4x2_ospfb_128/fft_wideband_real/fft_unscrambler/square_transposer/db1 ==
  din : Inport
  dly : xbsIndex_r4/Delay  rst=off  infoeditControl=Selection of Reset will increase slice count due to use of real FFs and instead of SRLs  en=off  latency=DelayLen  reg_retiming=on  dbl_ovrd=off  block_type=delay
  dout : Outport
  wires:
  din/1 -> dly/1
  dly/1 -> dout/1

== system rfsoc4x2_ospfb_128/fft_wideband_real/fft_unscrambler/square_transposer/db2 ==
  din : Inport
  dly : xbsIndex_r4/Delay  rst=off  infoeditControl=Selection of Reset will increase slice count due to use of real FFs and instead of SRLs  en=off  latency=DelayLen  reg_retiming=on  dbl_ovrd=off  block_type=delay
  dout : Outport
  wires:
  din/1 -> dly/1
  dly/1 -> dout/1

== system rfsoc4x2_ospfb_128/fft_wideband_real/fft_unscrambler/square_transposer/db3 ==
  din : Inport
  dly : xbsIndex_r4/Delay  rst=off  infoeditControl=Selection of Reset will increase slice count due to use of real FFs and instead of SRLs  en=off  latency=DelayLen  reg_retiming=on  dbl_ovrd=off  block_type=delay
  dout : Outport
  wires:
  din/1 -> dly/1
  dly/1 -> dout/1

== system rfsoc4x2_ospfb_128/fft_wideband_real/fft_unscrambler/square_transposer/db4 ==
  din : Inport
  dly : xbsIndex_r4/Delay  rst=off  infoeditControl=Selection of Reset will increase slice count due to use of real FFs and instead of SRLs  en=off  latency=DelayLen  reg_retiming=on  dbl_ovrd=off  block_type=delay
  dout : Outport
  wires:
  din/1 -> dly/1
  dly/1 -> dout/1

== system rfsoc4x2_ospfb_128/fft_wideband_real/fft_unscrambler/square_transposer/db5 ==
  din : Inport
  dly : xbsIndex_r4/Delay  rst=off  infoeditControl=Selection of Reset will increase slice count due to use of real FFs and instead of SRLs  en=off  latency=DelayLen  reg_retiming=on  dbl_ovrd=off  block_type=delay
  dout : Outport
  wires:
  din/1 -> dly/1
  dly/1 -> dout/1

== system rfsoc4x2_ospfb_128/fft_wideband_real/fft_unscrambler/square_transposer/db6 ==
  din : Inport
  dly : xbsIndex_r4/Delay  rst=off  infoeditControl=Selection of Reset will increase slice count due to use of real FFs and instead of SRLs  en=off  latency=DelayLen  reg_retiming=on  dbl_ovrd=off  block_type=delay
  dout : Outport
  wires:
  din/1 -> dly/1
  dly/1 -> dout/1

== system rfsoc4x2_ospfb_128/fft_wideband_real/fft_unscrambler/square_transposer/df1 ==
  din : Inport
  dly : xbsIndex_r4/Delay  rst=off  infoeditControl=Selection of Reset will increase slice count due to use of real FFs and instead of SRLs  en=off  latency=DelayLen  reg_retiming=on  dbl_ovrd=off  block_type=delay
  dout : Outport
  wires:
  din/1 -> dly/1
  dly/1 -> dout/1

== system rfsoc4x2_ospfb_128/fft_wideband_real/fft_unscrambler/square_transposer/df2 ==
  din : Inport
  dly : xbsIndex_r4/Delay  rst=off  infoeditControl=Selection of Reset will increase slice count due to use of real FFs and instead of SRLs  en=off  latency=DelayLen  reg_retiming=on  dbl_ovrd=off  block_type=delay
  dout : Outport
  wires:
  din/1 -> dly/1
  dly/1 -> dout/1

== system rfsoc4x2_ospfb_128/fft_wideband_real/fft_unscrambler/square_transposer/df3 ==
  din : Inport
  dly : xbsIndex_r4/Delay  rst=off  infoeditControl=Selection of Reset will increase slice count due to use of real FFs and instead of SRLs  en=off  latency=DelayLen  reg_retiming=on  dbl_ovrd=off  block_type=delay
  dout : Outport
  wires:
  din/1 -> dly/1
  dly/1 -> dout/1

== system rfsoc4x2_ospfb_128/fft_wideband_real/fft_unscrambler/square_transposer/df4 ==
  din : Inport
  dly : xbsIndex_r4/Delay  rst=off  infoeditControl=Selection of Reset will increase slice count due to use of real FFs and instead of SRLs  en=off  latency=DelayLen  reg_retiming=on  dbl_ovrd=off  block_type=delay
  dout : Outport
  wires:
  din/1 -> dly/1
  dly/1 -> dout/1

== system rfsoc4x2_ospfb_128/fft_wideband_real/fft_unscrambler/square_transposer/df5 ==
  din : Inport
  dly : xbsIndex_r4/Delay  rst=off  infoeditControl=Selection of Reset will increase slice count due to use of real FFs and instead of SRLs  en=off  latency=DelayLen  reg_retiming=on  dbl_ovrd=off  block_type=delay
  dout : Outport
  wires:
  din/1 -> dly/1
  dly/1 -> dout/1

== system rfsoc4x2_ospfb_128/fft_wideband_real/fft_unscrambler/square_transposer/df6 ==
  din : Inport
  dly : xbsIndex_r4/Delay  rst=off  infoeditControl=Selection of Reset will increase slice count due to use of real FFs and instead of SRLs  en=off  latency=DelayLen  reg_retiming=on  dbl_ovrd=off  block_type=delay
  dout : Outport
  wires:
  din/1 -> dly/1
  dly/1 -> dout/1

== system rfsoc4x2_ospfb_128/fft_wideband_real/fft_unscrambler/square_transposer/df7 ==
  din : Inport
  dly : xbsIndex_r4/Delay  rst=off  infoeditControl=Selection of Reset will increase slice count due to use of real FFs and instead of SRLs  en=off  latency=DelayLen  reg_retiming=on  dbl_ovrd=off  block_type=delay
  dout : Outport
  wires:
  din/1 -> dly/1
  dly/1 -> dout/1

== system rfsoc4x2_ospfb_128/fft_wideband_real/fft_unscrambler/square_transposer/dsync ==
  din : Inport
  dly : xbsIndex_r4/Delay  rst=off  infoeditControl=Selection of Reset will increase slice count due to use of real FFs and instead of SRLs  en=off  latency=DelayLen  reg_retiming=on  dbl_ovrd=off  block_type=delay
  dout : Outport
  wires:
  din/1 -> dly/1
  dly/1 -> dout/1
